simulink subsystem "Shadow"  (R2024b)
settings: Solver=VariableStepAuto  StartTime=0.0  StopTime=10.0  RelTol=1e-3
libraries: simulink x1
settings Model: Creator=marco  LastModifiedBy=ferru

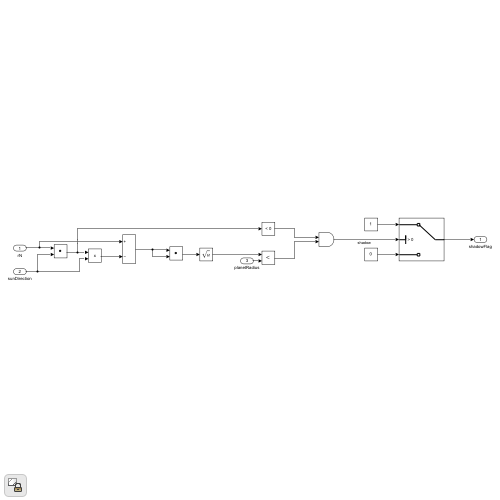
[thumbnail: Simulink's stored preview of the top-level diagram]
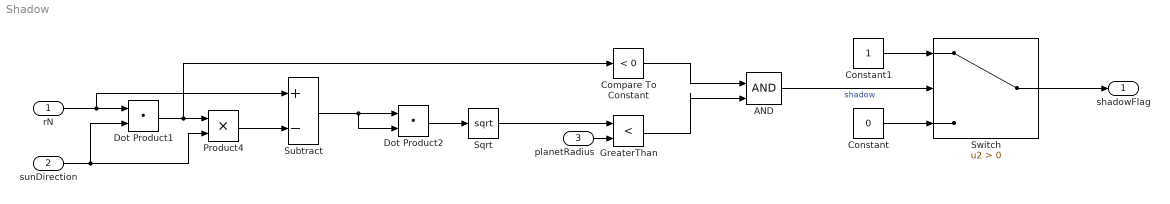
== system Shadow ==
  rN : Inport
  sunDirection : Inport  Port=2
  planetRadius : Inport  Port=3
  AND : Logic  IconShape=distinctive  AllPortsSameDT=off  OutDataTypeStr=boolean
  Compare To Constant : simulink/Logic and Bit Operations/Compare To Constant  relop=<  const=0  OutDataTypeStr=boolean
  Constant : Constant  Value=0
  Constant1 : Constant
  Dot Product1 : DotProduct  OutDataTypeStr=Inherit: Inherit via internal rule
  Dot Product2 : DotProduct  OutDataTypeStr=Inherit: Inherit via internal rule
  GreaterThan : RelationalOperator  Operator=<  OutDataTypeStr=boolean  RndMeth=Simplest  InputSameDT=off
  Product4 : Product
  Sqrt : Sqrt
  Subtract : Sum  Inputs=+-
  Switch : Switch  Criteria=u2 > Threshold  SaturateOnIntegerOverflow=off  InputSameDT=off
  shadowFlag : Outport
  wires:
  sunDirection/1 -> Dot Product1/2, Product4/2
  Dot Product2/1 -> Sqrt/1
  Dot Product1/1 -> Product4/1, Compare To Constant/1
  GreaterThan/1 -> AND/2
  rN/1 -> Dot Product1/1, Subtract/1
  Product4/1 -> Subtract/2
  Constant/1 -> Switch/3
  AND/1 -> Switch/2  "shadow"
  Subtract/1 -> Dot Product2/1, Dot Product2/2
  Constant1/1 -> Switch/1
  Compare To Constant/1 -> AND/1
  Sqrt/1 -> GreaterThan/1
  Switch/1 -> shadowFlag/1
  planetRadius/1 -> GreaterThan/2
